simulink model "boost_converter_openloop"  (R2026a)
settings: Solver=ode15s  StopTime=0.1  RelTol=1e-6  AbsTol=1e-9
undefined symbols (not defined in the file): C, D, L, rL, Rload, Vin
settings Model: Creator=akash  LastModifiedBy=akash

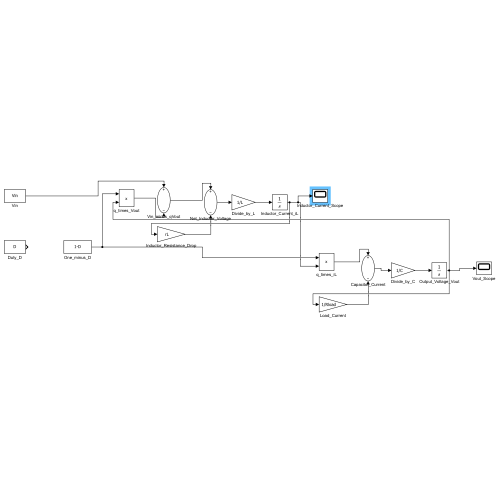
[thumbnail: Simulink's stored preview of the top-level diagram]
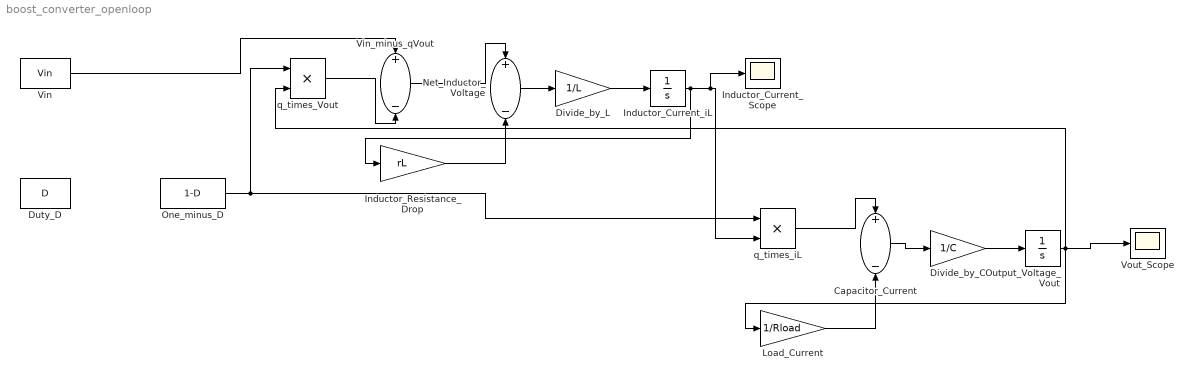
== system boost_converter_openloop ==
  Capacitor_Current : Sum  Inputs=+-
  Divide_by_C : Gain  Gain=1/C
  Divide_by_L : Gain  Gain=1/L
  Duty_D : Constant  Value=D
  Inductor_Current_Scope : Scope
      settings: ActiveDisplayYMinimum=-38.450921766107022  ActiveDisplayYMaximum=55.537704920728906
  Inductor_Current_iL : Integrator
  Inductor_Resistance_Drop : Gain  Gain=rL
  Load_Current : Gain  Gain=1/Rload
  Net_Inductor_Voltage : Sum  Inputs=+-
  One_minus_D : Constant  Value=1-D
  Output_Voltage_Vout : Integrator
  Vin : Constant  Value=Vin
  Vin_minus_qVout : Sum  Inputs=+-
  Vout_Scope : Scope
      settings: ActiveDisplayYMinimum=-25.981043402684818  ActiveDisplayYMaximum=226.19613654816297
  q_times_Vout : Product  Inputs=**
  q_times_iL : Product  Inputs=**
  wires:
  One_minus_D/1 -> q_times_Vout/1, q_times_iL/1
  Output_Voltage_Vout/1 -> q_times_Vout/2, Load_Current/1, Vout_Scope/1
  Vin/1 -> Vin_minus_qVout/1
  q_times_Vout/1 -> Vin_minus_qVout/2
  Inductor_Current_iL/1 -> q_times_iL/2, Inductor_Current_Scope/1, Inductor_Resistance_Drop/1
  Vin_minus_qVout/1 -> Net_Inductor_Voltage/1
  Inductor_Resistance_Drop/1 -> Net_Inductor_Voltage/2
  Net_Inductor_Voltage/1 -> Divide_by_L/1
  Divide_by_L/1 -> Inductor_Current_iL/1
  q_times_iL/1 -> Capacitor_Current/1
  Load_Current/1 -> Capacitor_Current/2
  Capacitor_Current/1 -> Divide_by_C/1
  Divide_by_C/1 -> Output_Voltage_Vout/1
